simulink model "Boost_24V_28V_equiv_v1"  (R2021b)
settings: Solver=FixedStepDiscrete  StartTime=0.0  StopTime=p_tStop  FixedStep=p_Ts  RelTol=1e-3
model workspace (MAT data in the model file):
  p_C = 4e-05
  p_D = 0.1640625
  p_ESR = 0.01
  p_IL0 = 1.66962699822
  p_L = 2.2e-05
  p_RL = 0.074
  p_Rdiode = 0.001
  p_Rload = 14
  p_Ron = 0.06
  p_Ts = 1.63578308208e-08
  p_Vc0 = 23.3747779751
  p_Vf = 0.5
  p_Vin = 24
  p_fsw = 477600
  p_pwmStart = 0.003
  p_pwmSteps = 128
  p_softStart = 0.005
  p_tStop = 0.02
libraries: spsSeriesRLCBranchLib x3, simulink x2, spsCurrentMeasurementLib x2, spsVoltageMeasurementLib x2, spsDiodeLib x1, spsGroundLib x1, spsIdealSwitchLib x1, spsDCVoltageSourceLib x1, spspowerguiLib x1
settings Model: Creator=Project contributors  LastModifiedBy=Project contributors
settings DataIOCC: SaveOutput=off  SignalLogging=off  SaveTime=off

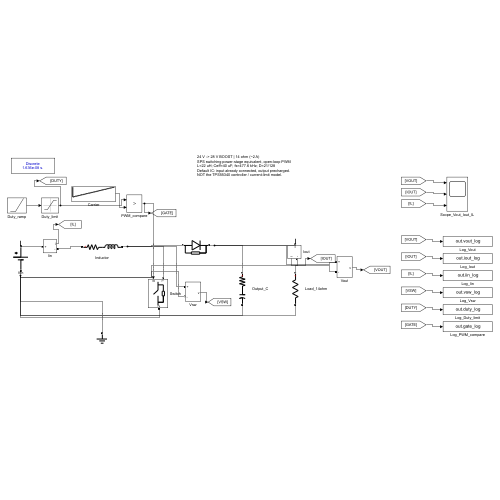
[thumbnail: Simulink's stored preview of the top-level diagram]
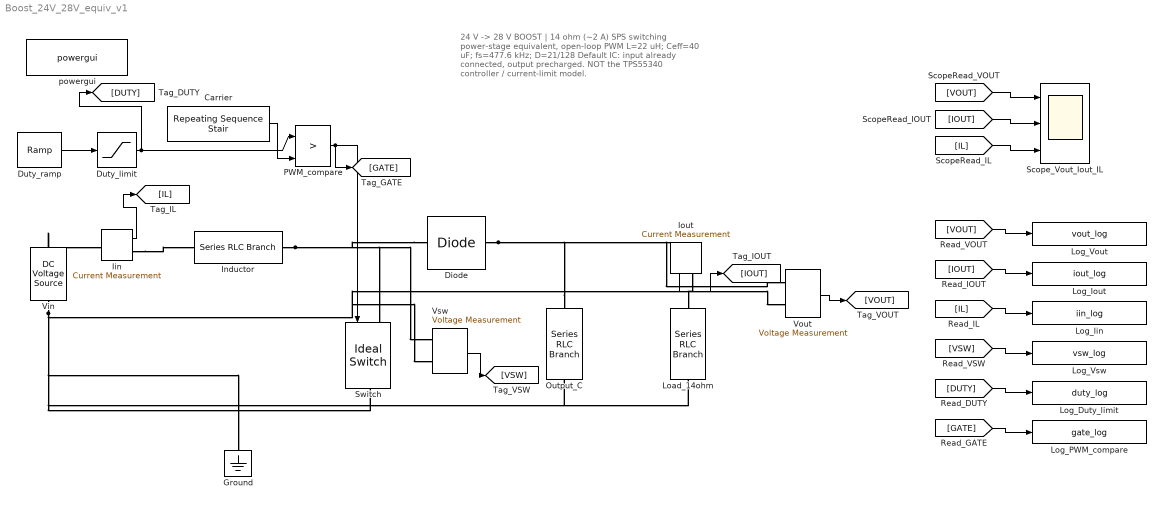
== system Boost_24V_28V_equiv_v1 ==
  note: 24 V -> 28 V BOOST | 14 ohm (~2 A)
      | SPS switching power-stage equivalent, open-loop PWM
      | L=22 uH; Ceff=40 uF; fs=477.6 kHz; D=21/128
      | Default IC: input already connected, output precharged.
      | NOT the TPS55340 controller / current-limit model.
  Carrier : simulink/Sources/Repeating Sequence Stair  OutValues=((0:p_pwmSteps-1)+0.5)/p_pwmSteps  tsamp=p_Ts  OutMin=[]  OutMax=[]  OutDataTypeStr=double  OutputDataTypeScalingMode=double  OutDataType=fixdt(0,8)  ConRadixGroup=Best Precision: Vector-wise  OutScaling=2^-12
  Diode : spsDiodeLib/Diode  Ron=p_Rdiode  Lon=0  Vf=p_Vf  IC=0  UseSnubber=0  Rs=500  Cs=250e-9  Measurements=off
  Duty_limit : Saturate  UpperLimit=p_D  LowerLimit=0
  Duty_ramp : simulink/Sources/Ramp  slope=p_D/p_softStart  start=p_pwmStart  InitialOutput=0
  Ground : spsGroundLib/Ground  LConnTagsString=a
  Iin : spsCurrentMeasurementLib/Current Measurement  PhasorSimulation=off  OutputType=Complex  PSBequivalent=0
  Inductor : spsSeriesRLCBranchLib/Series RLC Branch  LConnTagsString=__new0  RConnTagsString=__new0  BranchType=RL  Resistance=p_RL  Inductance=p_L  SetiL0=on  InitialCurrent=p_IL0  Capacitance=1e-6  Setx0=off  InitialVoltage=0  Measurements=None
  Iout : spsCurrentMeasurementLib/Current Measurement  PhasorSimulation=off  OutputType=Complex  PSBequivalent=0
  Load_14ohm : spsSeriesRLCBranchLib/Series RLC Branch  LConnTagsString=__new0  RConnTagsString=__new0  BranchType=R  Resistance=p_Rload  Inductance=1e-3  SetiL0=off  InitialCurrent=0  Capacitance=1e-6  Setx0=off  InitialVoltage=0  Measurements=None
  Log_Duty_limit : ToWorkspace  VariableName=duty_log  SaveFormat=Timeseries  SampleTime=-1
  Log_Iin : ToWorkspace  VariableName=iin_log  SaveFormat=Timeseries  SampleTime=-1
  Log_Iout : ToWorkspace  VariableName=iout_log  SaveFormat=Timeseries  SampleTime=-1
  Log_PWM_compare : ToWorkspace  VariableName=gate_log  SaveFormat=Timeseries  SampleTime=-1
  Log_Vout : ToWorkspace  VariableName=vout_log  SaveFormat=Timeseries  SampleTime=-1
  Log_Vsw : ToWorkspace  VariableName=vsw_log  SaveFormat=Timeseries  SampleTime=-1
  Output_C : spsSeriesRLCBranchLib/Series RLC Branch  LConnTagsString=__new0  RConnTagsString=__new0  BranchType=RC  Resistance=p_ESR  Inductance=1e-3  SetiL0=off  InitialCurrent=0  Capacitance=p_C  Setx0=on  InitialVoltage=p_Vc0  Measurements=None
  PWM_compare : RelationalOperator  Operator=>  OutDataTypeStr=boolean  RndMeth=Simplest
  Scope_Vout_Iout_IL : Scope  NumInputPorts=3
  Switch : spsIdealSwitchLib/Ideal Switch  Ron=p_Ron  Lon=0  IC=0  Rs=1e6  Cs=inf  Measurements=off
  Vin : spsDCVoltageSourceLib/DC Voltage Source  Amplitude=p_Vin  Measurements=None
  Vout : spsVoltageMeasurementLib/Voltage Measurement  PhasorSimulation=off  OutputType=Complex  PSBequivalent=0
  Vsw : spsVoltageMeasurementLib/Voltage Measurement  PhasorSimulation=off  OutputType=Complex  PSBequivalent=0
  powergui : spspowerguiLib/powergui  Priority=1  SimulationMode=Discrete  SampleTime=p_Ts  frequency=60  Iterations=50  frequencyindice=60  Pbase=100e6  ErrMax=1e-4  UnitsV=kV  UnitsW=MW  buscounter=0  FunctionMessages=off  echomessages=off  EnableUseOfTLC=off  CurrentSourceSwitches=off  DisableSnubberDevices=off  DisableRonSwitches=off  DisableVfSwitches=off  DisplayEquations=off  AutomaticDiscreteSolvers=off  SolverType=Tustin/Backward Euler (TBE)  Interpol=off  ExternalGateDelay=off  methode=off  Ts=100  x0status=blocks  SPID=on  SwTol=0  HookPort=off  NonlinearTolerance=1e-4  nMaxIteration=100  ContinueOnMaxIteration=off  RestoreLinks=warning  ResistiveCurrentMeasurement=off  Frange=[0:2:500]  Ylog=off  Xlog=on  ShowGrid=off  save=off  variable=ZData  structure=0  ZoomFFT=off  StartTime=0.0  cycles=1  DisplayStyle=1  fundamental=60  FreqAxis=off  MaxFrequency=1000  frequencyindicesteady=1  RmsSteady=1  display=off
  wires:
  Duty_ramp/1 -> Duty_limit/1
  Duty_limit/1 -> PWM_compare/1, [DUTY]
  Carrier/1 -> PWM_compare/2
  PWM_compare/1 -> Switch/1, [GATE]
  Vout/1 -> [VOUT]
  [VOUT] -> Log_Vout/1
  [VOUT] -> Scope_Vout_Iout_IL/1
  Iout/1 -> [IOUT]
  [IOUT] -> Log_Iout/1
  [IOUT] -> Scope_Vout_Iout_IL/2
  Iin/1 -> [IL]
  [IL] -> Log_Iin/1
  [IL] -> Scope_Vout_Iout_IL/3
  Vsw/1 -> [VSW]
  [VSW] -> Log_Vsw/1
  [DUTY] -> Log_Duty_limit/1
  [GATE] -> Log_PWM_compare/1
  connections:
  Vin/RConn1 -- Iin/LConn1
  Iin/RConn1 -- Inductor/LConn1
  Diode/LConn1 -- Inductor/RConn1 -- Switch/LConn1 -- Vsw/LConn1
  Output_C/LConn1 -- Diode/RConn1 -- Iout/LConn1 -- Vout/LConn1
  Iout/RConn1 -- Load_14ohm/LConn1
  Switch/RConn1 -- Vin/LConn1 -- Output_C/RConn1 -- Load_14ohm/RConn1 -- Vout/LConn2 -- Vsw/LConn2 -- Ground/LConn1
